simulink model "s_b4a4x4kf"  (R2018a)
settings: Solver=VariableStepDiscrete  StartTime=0.0  StopTime=1  RelTol=1e-3
undefined symbols (not defined in the file): fft_stages, n_bits_ants, n_bits_xengs
libraries: xbsIndex_r4 x22457, casper_library_misc x31, xbsReplacements_r4 x30, casper_library_scopes x17, xps_library x4
(part 141 of 232)

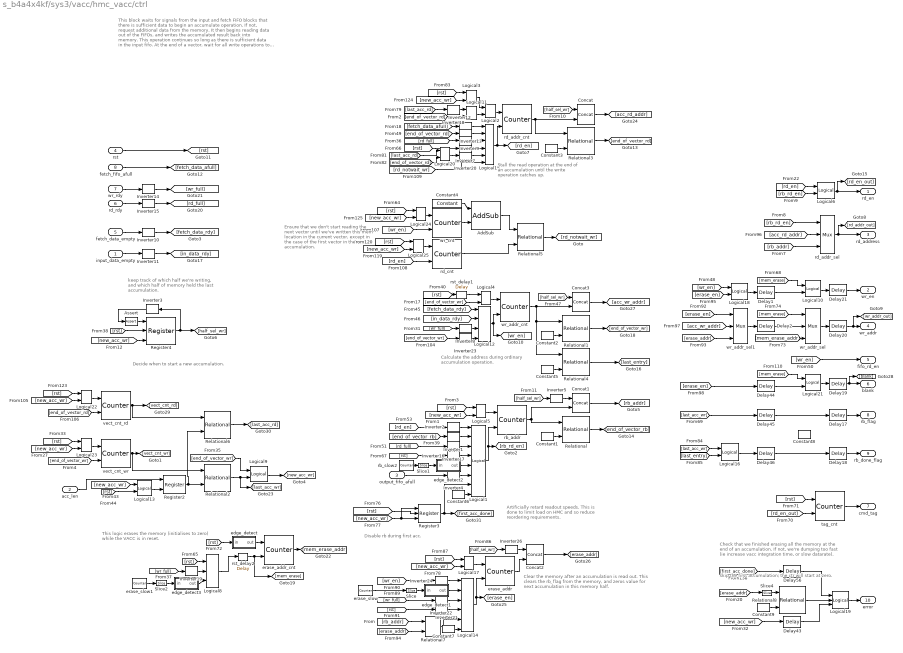
== system s_b4a4x4kf/sys3/vacc/hmc_vacc/ctrl ==
  note: Clear the memory after an accumulation is read out.
      | This clears the rb_flag from the memory, and
      | zeros value for next accumulation in this memory half.
  note: Stall the read operation
      | at the end of an accumulation
      | until the write operation catches up.
  note: Ensure that we don't start reading
      | the next vector until we've written
      | this mem location in the current vector,
      | except in the case of the first vector in
      | the accumulation.
  note: Disable rb during first acc.
  note: Artificially retard readout speeds.
      | This is done to limit load on HMC and
      | so reduce reordering requirements.
  note: This logic erases the memory (initialises to zero)
      | while the VACC is in reset.
  note: Decide when to start a new accumulation.
  note: Calculate the address during ordinary
      | accumulation operation.
  note: keep track of which half we're writing,
      | and which half of memory
      | held the last accumulation.
  note: This block waits for signals from the
      | input and fetch FIFO blocks that there is sufficient data
      | to begin an accumulate operation.
      |
      | If not, request additional data from the memory.
      |
      | It then begins reading data out of the FIFOs, and writes the
      | accumulated result back into memory.
      |
      | This operation continues so long as there is
      | sufficient data in the input fifo.
      |
      | At the end of a vector, wait for all write operations
      | to finish before starting the next vector.
      |
      | Simultaneously, read back the previous integration during
      | unused rd/write operations. After reading a previous accumulated
      | value, try to clear that memory location.
  note: Check that we finished erasing all the memory
      | at the end of an accumulation.
      | If not, we're dumping too fast
      | (ie increase vacc integration time, or slow datarate).
  note: skip the first accumulation; the ctr will start at zero.
  input_data_empty : Inport
  acc_len : Inport  Port=2
  output_fifo_afull : Inport  Port=3
  rst : Inport  Port=4
  fetch_data_empty : Inport  Port=5
  rd_rdy : Inport  Port=6
  wr_rdy : Inport  Port=7
  fetch_fifo_afull : Inport  Port=8
  AddSub : xbsIndex_r4/AddSub  mode=Addition  use_carryin=off  use_carryout=off  en=off  latency=1  precision=Full  arith_type=Unsigned  n_bits=16  bin_pt=14  quantization=Truncate  overflow=Wrap  use_behavioral_HDL=off  hw_selection=Fabric  pipelined=off  dbl_ovrd=off  block_type=addsub
  Assert : xbsIndex_r4/Assert  assert_type=on  type_source=Explicitly  gui_display_data_type=Fixed-point  arith_type=Unsigned  n_bits=1  bin_pt=0  preci_type=Single  exp_width=8  frac_width=24  assert_rate=on  rate_source=Explicitly  period=1  output_port=on  block_type=assert
      settings: infoedit=Asserts a user-defined sample rate and/or type on a signal.<P><P>Hardware notes: In hardware this block costs nothing.  block_version=10.1.3
  Concat{,1..3} (4 alike) : xbsIndex_r4/Concat  num_inputs=2  dbl_ovrd=off  block_type=concat
      settings: block_version=10.1.3
  Constant{1..3,9} (4 alike) : xbsIndex_r4/Constant  const=vector_len  gui_display_data_type=Fixed-point  arith_type=Unsigned  n_bits=vector_bits  bin_pt=0  preci_type=Single  exp_width=8  frac_width=24  explicit_period=on  period=1  equ=P=C  opselect=C  inp2=PCIN>>17  opr=+  inp1=P  carry=CIN  dbl_ovrd=off  block_type=constant
  Constant4 : xbsIndex_r4/Constant  const=vector_len-4  gui_display_data_type=Fixed-point  arith_type=Unsigned  n_bits=vector_bits  bin_pt=0  preci_type=Single  exp_width=8  frac_width=24  explicit_period=on  period=1  equ=P=C  opselect=C  inp2=PCIN>>17  opr=+  inp1=P  carry=CIN  dbl_ovrd=off  block_type=constant
  Constant5 : xbsIndex_r4/Constant  const=vector_len-1  gui_display_data_type=Fixed-point  arith_type=Unsigned  n_bits=vector_bits  bin_pt=0  preci_type=Single  exp_width=8  frac_width=24  explicit_period=on  period=1  equ=P=C  opselect=C  inp2=PCIN>>17  opr=+  inp1=P  carry=CIN  dbl_ovrd=off  block_type=constant
  Constant6 : xbsIndex_r4/Constant  const=1  gui_display_data_type=Boolean  arith_type=Boolean  n_bits=1  bin_pt=0  preci_type=Single  exp_width=8  frac_width=24  explicit_period=on  period=1  equ=P=C  opselect=C  inp2=PCIN>>17  opr=+  inp1=P  carry=CIN  dbl_ovrd=off  block_type=constant
  Constant7 : xbsIndex_r4/Constant  const=1  gui_display_data_type=Boolean  arith_type=Boolean  n_bits=1  bin_pt=0  preci_type=Single  exp_width=8  frac_width=24  explicit_period=on  period=1  equ=P=C  opselect=C  inp2=PCIN>>17  opr=+  inp1=P  carry=CIN  dbl_ovrd=off  block_type=constant
  Constant8 : xbsIndex_r4/Constant  const=0  gui_display_data_type=Boolean  arith_type=Boolean  n_bits=1  bin_pt=0  preci_type=Single  exp_width=8  frac_width=24  explicit_period=on  period=1  equ=P=C  opselect=C  inp2=PCIN>>17  opr=+  inp1=P  carry=CIN  dbl_ovrd=off  block_type=constant
  Delay{1..2,44..46} (5 alike) : xbsIndex_r4/Delay  rst=off  infoeditControl=Selection of Reset will increase slice count due to use of real FFs and instead of SRLs  en=off  latency=delay_fifo  reg_retiming=on  dbl_ovrd=off  block_type=delay
      settings: infoedit=Hardware notes: A delay line is a chain, each link of which is an SRL16 or SRL32 followed by a flip-flop.
  Delay{17..21} (5 alike) : xbsIndex_r4/Delay  rst=off  infoeditControl=Selection of Reset will increase slice count due to use of real FFs and instead of SRLs  en=off  latency=delay_adder  reg_retiming=on  dbl_ovrd=off  block_type=delay
      settings: infoedit=Hardware notes: A delay line is a chain, each link of which is an SRL16 or SRL32 followed by a flip-flop.
  Delay43 : xbsIndex_r4/Delay  rst=off  infoeditControl=Selection of Reset will increase slice count due to use of real FFs and instead of SRLs  en=off  latency=1  reg_retiming=on  dbl_ovrd=off  block_type=delay
      settings: infoedit=Hardware notes: A delay line is a chain, each link of which is an SRL16 or SRL32 followed by a flip-flop.
  Delay56 : xbsIndex_r4/Delay  rst=off  infoeditControl=Selection of Reset will increase slice count due to use of real FFs and instead of SRLs  en=off  latency=1  reg_retiming=on  dbl_ovrd=off  block_type=delay
      settings: infoedit=Hardware notes: A delay line is a chain, each link of which is an SRL16 or SRL32 followed by a flip-flop.
  Inverter{1..5,7..24,26} (24 alike) : xbsIndex_r4/Inverter  en=off  latency=0  dbl_ovrd=off  block_type=inv
  Logical1 : xbsIndex_r4/Logical  logical_function=AND  inputs=8  en=off  latency=0  precision=Full  arith_type=Unsigned  n_bits=16  bin_pt=0  align_bp=on  dbl_ovrd=off  block_type=logical
  Logical{2..6,10,13,17..18,21..25} (14 alike) : xbsIndex_r4/Logical  logical_function=OR  inputs=2  en=off  latency=0  precision=Full  arith_type=Unsigned  n_bits=16  bin_pt=0  align_bp=on  dbl_ovrd=off  block_type=logical
  Logical{9,11,16,20} (4 alike) : xbsIndex_r4/Logical  logical_function=AND  inputs=2  en=off  latency=0  precision=Full  arith_type=Unsigned  n_bits=16  bin_pt=0  align_bp=on  dbl_ovrd=off  block_type=logical
  Logical12 : xbsIndex_r4/Logical  logical_function=AND  inputs=4  en=off  latency=0  precision=Full  arith_type=Unsigned  n_bits=16  bin_pt=0  align_bp=on  dbl_ovrd=off  block_type=logical
  Logical14 : xbsIndex_r4/Logical  logical_function=AND  inputs=6  en=off  latency=0  precision=Full  arith_type=Unsigned  n_bits=16  bin_pt=0  align_bp=on  dbl_ovrd=off  block_type=logical
  Logical15 : xbsIndex_r4/Logical  logical_function=AND  inputs=6  en=off  latency=0  precision=Full  arith_type=Unsigned  n_bits=16  bin_pt=0  align_bp=on  dbl_ovrd=off  block_type=logical
  Logical19 : xbsIndex_r4/Logical  logical_function=AND  inputs=3  en=off  latency=0  precision=Full  arith_type=Unsigned  n_bits=16  bin_pt=0  align_bp=on  dbl_ovrd=off  block_type=logical
  Logical8 : xbsIndex_r4/Logical  logical_function=AND  inputs=3  en=off  latency=0  precision=Full  arith_type=Unsigned  n_bits=16  bin_pt=0  align_bp=on  dbl_ovrd=off  block_type=logical
  Register2 : xbsIndex_r4/Register  init=0  rst=off  en=on  dbl_ovrd=off  block_type=register
  Register3 : xbsIndex_r4/Register  init=0  rst=on  en=on  dbl_ovrd=off  block_type=register
  Register4 : xbsIndex_r4/Register  init=0  rst=on  en=on  dbl_ovrd=off  block_type=register
  Relational{,1..4,6} (6 alike) : xbsIndex_r4/Relational  mode=a>=b  op_type=Bool  en=off  latency=0  dbl_ovrd=off  block_type=relational
      settings: block_version=10.1.3
  Relational5 : xbsIndex_r4/Relational  mode=a>b  op_type=Bool  en=off  latency=1  dbl_ovrd=off  block_type=relational
      settings: block_version=10.1.3
  Relational7 : xbsIndex_r4/Relational  mode=a>b  op_type=Bool  en=off  latency=0  dbl_ovrd=off  block_type=relational
      settings: block_version=10.1.3
  Relational8 : xbsIndex_r4/Relational  mode=a!=b  op_type=Bool  en=off  latency=1  dbl_ovrd=off  block_type=relational
      settings: block_version=10.1.3
  Slice : xbsIndex_r4/Slice  nbits=1  boolean_output=on  mode=Upper Bit Location + Width  bit1=0  base1=MSB of Input  bit0=0  base0=LSB of Input  dbl_ovrd=off  block_type=slice
  Slice1 : xbsIndex_r4/Slice  nbits=1  boolean_output=on  mode=Upper Bit Location + Width  bit1=0  base1=MSB of Input  bit0=0  base0=LSB of Input  dbl_ovrd=off  block_type=slice
  Slice2 : xbsIndex_r4/Slice  nbits=1  boolean_output=on  mode=Upper Bit Location + Width  bit1=0  base1=MSB of Input  bit0=0  base0=LSB of Input  dbl_ovrd=off  block_type=slice
  Slice4 : xbsIndex_r4/Slice  nbits=1  boolean_output=off  mode=Two Bit Locations  bit1=-1  base1=MSB of Input  bit0=0  base0=LSB of Input  dbl_ovrd=off  block_type=slice
  edge_detect : Subsystem  mask(edge_detect){edge=Rising, polarity=Active High, x_in=[0 0.08 0.08 0.16 0.16 0.24 0.24 0.32 0.32 0.4], y_in=[-1 -1  1  1  1  1  1  1  1  1], x_out=[0.6 0.68 0.68 0.76 0.76 0.84 0.84 0.92 0.92 1], y_out=[-1 -1  1  1 -1 -1 -1 -1 -1 -1]}
      mask prompts: edge "Edge Type"; polarity "Output Polarity"; x_in "Input X Positions"; y_in "Input Y Positions"; x_out "Output X Positions"; y_out "Output Y Positions"
      mask help: Output is active for one-cycle after each edge of the specified type (i.e. rising, falling or both).
      mask init: same as s_b4a4x4kf/edge_detect
      settings: AttributesFormatString=|
      | rising edges
      | active high
      mask Help: Output is active for one-cycle after each edge of the specified type (i.e. rising, falling, or both).  Latency is zero.
      mask TypeOptions edge: Rising | Falling | Both
      mask TypeOptions polarity: Active High | Active Low
      mask Display:
      | plot(x_in_num,0.5+y_in_num*0.2);
      | plot(x_out_num,0.5+y_out_num*0.2);
  edge_detect1 : Subsystem  mask(edge_detect){edge=Rising, polarity=Active High, x_in=[0 0.08 0.08 0.16 0.16 0.24 0.24 0.32 0.32 0.4], y_in=[-1 -1  1  1  1  1  1  1  1  1], x_out=[0.6 0.68 0.68 0.76 0.76 0.84 0.84 0.92 0.92 1], y_out=[-1 -1  1  1 -1 -1 -1 -1 -1 -1]}
      mask prompts: edge "Edge Type"; polarity "Output Polarity"; x_in "Input X Positions"; y_in "Input Y Positions"; x_out "Output X Positions"; y_out "Output Y Positions"
      mask help: Output is active for one-cycle after each edge of the specified type (i.e. rising, falling or both).
      mask init: same as s_b4a4x4kf/edge_detect
      settings: AttributesFormatString=|
      | rising edges
      | active high
      mask Help: Output is active for one-cycle after each edge of the specified type (i.e. rising, falling, or both).  Latency is zero.
      mask TypeOptions edge: Rising | Falling | Both
      mask TypeOptions polarity: Active High | Active Low
      mask Display:
      | plot(x_in_num,0.5+y_in_num*0.2);
      | plot(x_out_num,0.5+y_out_num*0.2);
  edge_detect2 : Subsystem  mask(edge_detect){edge=Rising, polarity=Active High, x_in=[0 0.08 0.08 0.16 0.16 0.24 0.24 0.32 0.32 0.4], y_in=[-1 -1  1  1  1  1  1  1  1  1], x_out=[0.6 0.68 0.68 0.76 0.76 0.84 0.84 0.92 0.92 1], y_out=[-1 -1  1  1 -1 -1 -1 -1 -1 -1]}
      mask prompts: edge "Edge Type"; polarity "Output Polarity"; x_in "Input X Positions"; y_in "Input Y Positions"; x_out "Output X Positions"; y_out "Output Y Positions"
      mask help: Output is active for one-cycle after each edge of the specified type (i.e. rising, falling or both).
      mask init: same as s_b4a4x4kf/edge_detect
      settings: AttributesFormatString=|
      | rising edges
      | active high
      mask Help: Output is active for one-cycle after each edge of the specified type (i.e. rising, falling, or both).  Latency is zero.
      mask TypeOptions edge: Rising | Falling | Both
      mask TypeOptions polarity: Active High | Active Low
      mask Display:
      | plot(x_in_num,0.5+y_in_num*0.2);
      | plot(x_out_num,0.5+y_out_num*0.2);
  edge_detect3 : Subsystem  mask(edge_detect){edge=Rising, polarity=Active High, x_in=[0 0.08 0.08 0.16 0.16 0.24 0.24 0.32 0.32 0.4], y_in=[-1 -1  1  1  1  1  1  1  1  1], x_out=[0.6 0.68 0.68 0.76 0.76 0.84 0.84 0.92 0.92 1], y_out=[-1 -1  1  1 -1 -1 -1 -1 -1 -1]}
      mask prompts: edge "Edge Type"; polarity "Output Polarity"; x_in "Input X Positions"; y_in "Input Y Positions"; x_out "Output X Positions"; y_out "Output Y Positions"
      mask help: Output is active for one-cycle after each edge of the specified type (i.e. rising, falling or both).
      mask init: same as s_b4a4x4kf/edge_detect
      settings: AttributesFormatString=|
      | rising edges
      | active high
      mask Help: Output is active for one-cycle after each edge of the specified type (i.e. rising, falling, or both).  Latency is zero.
      mask TypeOptions edge: Rising | Falling | Both
      mask TypeOptions polarity: Active High | Active Low
      mask Display:
      | plot(x_in_num,0.5+y_in_num*0.2);
      | plot(x_out_num,0.5+y_out_num*0.2);
  erase_addr : xbsIndex_r4/Counter  cnt_type=Free Running  cnt_to=Inf  operation=Up  start_count=0  cnt_by_val=1  arith_type=Unsigned  n_bits=vector_bits  bin_pt=0  load_pin=off  rst=on  en=on  explicit_period=on  period=1  use_behavioral_HDL=off  implementation=Fabric  use_rpm=off  dbl_ovrd=off  block_type=counter
  erase_addr_cnt : xbsIndex_r4/Counter  cnt_type=Free Running  cnt_to=vector_len-1  operation=Up  start_count=0  cnt_by_val=1  arith_type=Unsigned  n_bits=vector_bits+1  bin_pt=0  load_pin=off  rst=on  en=on  explicit_period=on  period=1  use_behavioral_HDL=off  implementation=Fabric  use_rpm=off  dbl_ovrd=off  block_type=counter
  erase_slow : xbsIndex_r4/Counter  cnt_type=Free Running  cnt_to=Inf  operation=Up  start_count=0  cnt_by_val=1  arith_type=Unsigned  n_bits=4  bin_pt=0  load_pin=off  rst=off  en=off  explicit_period=on  period=1  use_behavioral_HDL=on  implementation=Fabric  use_rpm=off  dbl_ovrd=off  block_type=counter
  erase_slow1 : xbsIndex_r4/Counter  cnt_type=Free Running  cnt_to=Inf  operation=Up  start_count=0  cnt_by_val=1  arith_type=Unsigned  n_bits=2  bin_pt=0  load_pin=off  rst=off  en=off  explicit_period=on  period=1  use_behavioral_HDL=on  implementation=Fabric  use_rpm=off  dbl_ovrd=off  block_type=counter
  rb_addr : xbsIndex_r4/Counter  cnt_type=Free Running  cnt_to=Inf  operation=Up  start_count=0  cnt_by_val=1  arith_type=Unsigned  n_bits=vector_bits  bin_pt=0  load_pin=off  rst=on  en=on  explicit_period=on  period=1  use_behavioral_HDL=off  implementation=Fabric  use_rpm=off  dbl_ovrd=off  block_type=counter
  rb_slow2 : xbsIndex_r4/Counter  cnt_type=Free Running  cnt_to=Inf  operation=Up  start_count=0  cnt_by_val=1  arith_type=Unsigned  n_bits=4  bin_pt=0  load_pin=off  rst=off  en=off  explicit_period=on  period=1  use_behavioral_HDL=on  implementation=Fabric  use_rpm=off  dbl_ovrd=off  block_type=counter
  rd_addr_cnt : xbsIndex_r4/Counter  cnt_type=Free Running  cnt_to=vector_len-1  operation=Up  start_count=0  cnt_by_val=1  arith_type=Unsigned  n_bits=vector_bits  bin_pt=0  load_pin=off  rst=on  en=on  explicit_period=on  period=1  use_behavioral_HDL=off  implementation=Fabric  use_rpm=off  dbl_ovrd=off  block_type=counter
  rd_addr_sel : xbsIndex_r4/Mux  inputs=2  en=off  latency=0  precision=Full  arith_type=Unsigned  n_bits=16  bin_pt=14  quantization=Truncate  overflow=Wrap  dbl_ovrd=off  block_type=mux
  rd_cnt : xbsIndex_r4/Counter  cnt_type=Free Running  cnt_to=vector_len-1  operation=Up  start_count=0  cnt_by_val=1  arith_type=Unsigned  n_bits=vector_bits+22  bin_pt=0  load_pin=off  rst=on  en=on  explicit_period=on  period=1  use_behavioral_HDL=off  implementation=Fabric  use_rpm=off  dbl_ovrd=off  block_type=counter
  rst_delay1 : xbsIndex_r4/Delay  rst=off  infoeditControl=Selection of Reset will increase slice count due to use of real FFs and instead of SRLs  en=off  latency=2  reg_retiming=on  dbl_ovrd=off  block_type=delay
  rst_delay2 : xbsIndex_r4/Delay  rst=off  infoeditControl=Selection of Reset will increase slice count due to use of real FFs and instead of SRLs  en=off  latency=1  reg_retiming=on  dbl_ovrd=off  block_type=delay
      settings: infoedit=Hardware notes: A delay line is a chain, each link of which is an SRL16 or SRL32 followed by a flip-flop.
  tag_cnt : xbsIndex_r4/Counter  cnt_type=Free Running  cnt_to=Inf  operation=Up  start_count=0  cnt_by_val=1  arith_type=Unsigned  n_bits=9  bin_pt=0  load_pin=off  rst=on  en=on  explicit_period=on  period=1  use_behavioral_HDL=off  implementation=Fabric  use_rpm=off  dbl_ovrd=off  block_type=counter
  vect_cnt_rd : xbsIndex_r4/Counter  cnt_type=Free Running  cnt_to=Inf  operation=Up  start_count=1  cnt_by_val=1  arith_type=Unsigned  n_bits=32  bin_pt=0  load_pin=off  rst=on  en=on  explicit_period=on  period=1  use_behavioral_HDL=off  implementation=Fabric  use_rpm=off  dbl_ovrd=off  block_type=counter
  vect_cnt_wr : xbsIndex_r4/Counter  cnt_type=Free Running  cnt_to=Inf  operation=Up  start_count=1  cnt_by_val=1  arith_type=Unsigned  n_bits=32  bin_pt=0  load_pin=off  rst=on  en=on  explicit_period=on  period=1  use_behavioral_HDL=off  implementation=Fabric  use_rpm=off  dbl_ovrd=off  block_type=counter
  wr_addr_cnt : xbsIndex_r4/Counter  cnt_type=Free Running  cnt_to=vector_len-1  operation=Up  start_count=0  cnt_by_val=1  arith_type=Unsigned  n_bits=vector_bits  bin_pt=0  load_pin=off  rst=on  en=on  explicit_period=on  period=1  use_behavioral_HDL=off  implementation=Fabric  use_rpm=off  dbl_ovrd=off  block_type=counter
  wr_addr_sel : xbsIndex_r4/Mux  inputs=2  en=off  latency=0  precision=Full  arith_type=Unsigned  n_bits=16  bin_pt=14  quantization=Truncate  overflow=Wrap  dbl_ovrd=off  block_type=mux
  wr_addr_sel1 : xbsIndex_r4/Mux  inputs=2  en=off  latency=0  precision=Full  arith_type=Unsigned  n_bits=16  bin_pt=14  quantization=Truncate  overflow=Wrap  dbl_ovrd=off  block_type=mux
  wr_cnt : xbsIndex_r4/Counter  cnt_type=Free Running  cnt_to=vector_len-1  operation=Up  start_count=0  cnt_by_val=1  arith_type=Unsigned  n_bits=vector_bits+22  bin_pt=0  load_pin=off  rst=on  en=on  explicit_period=on  period=1  use_behavioral_HDL=off  implementation=Fabric  use_rpm=off  dbl_ovrd=off  block_type=counter
  rd_en : Outport
  wr_en : Outport  Port=2
  rd_address : Outport  Port=3
  wr_addr : Outport  Port=4
  fifo_rd_en : Outport  Port=5
  blank : Outport  Port=6
  cmd_tag : Outport  Port=7
  rb_flag : Outport  Port=8
  rb_done_flag : Outport  Port=9
  error : Outport  Port=10
  wires:
  Concat1/1 -> [rb_addr]
  rb_addr/1 -> Concat1/2, Relational/1
  [rb_addr] -> rd_addr_sel/3
  Inverter5/1 -> Concat1/1
  [half_sel_wr] -> Inverter5/1
  [half_sel_wr] -> Concat/1
  Register2/1 -> Relational6/2, Relational2/2
  Logical9/1 -> [new_acc_wr]
  rst/1 -> [rst]
  Constant3/1 -> Relational3/2
  Assert/1 -> Register4/1
  Inverter3/1 -> Assert/1
  Register4/1 -> [half_sel_wr], Inverter3/1
  rd_addr_sel/1 -> rd_address/1, [rd_addr_out]
  [rb_rd_en] -> Logical6/2
  Concat/1 -> [acc_rd_addr]
  [rb_rd_en] -> rd_addr_sel/1
  Logical6/1 -> rd_en/1, [rd_en_out]
  Relational/1 -> [end_of_vector_rb]
  rd_addr_cnt/1 -> Relational3/1, Concat/2
  Logical15/1 -> rd_addr_cnt/2, [rd_en]
  [end_of_vector_wr] -> vect_cnt_wr/2
  Logical2/1 -> rd_addr_cnt/1
  Logical3/1 -> Logical2/1
  Relational2/1 -> [last_acc_wr], Logical9/2
  [end_of_vector_wr] -> Logical9/1
  Logical1/1 -> rb_addr/2, [rb_rd_en]
  [rst] -> Register4/2
  [rd_en] -> Inverter2/1
  [new_acc_wr] -> Logical13/1
  [rst] -> Logical13/2
  acc_len/1 -> Register2/1
  Logical13/1 -> Register2/2
  Logical4/1 -> wr_addr_cnt/1
  fetch_data_empty/1 -> Inverter10/1
  input_data_empty/1 -> Inverter11/1
  Inverter10/1 -> [fetch_data_rdy]
  Inverter11/1 -> [in_data_rdy]
  [fetch_data_afull] -> Inverter12/1
  [end_of_vector_rd] -> Inverter13/1
  Inverter12/1 -> Logical15/1
  Inverter13/1 -> Logical15/2
  Relational1/1 -> [end_of_vector_wr]
  Constant2/1 -> Relational1/2
  [end_of_vector_wr] -> Logical4/2
  [rst] -> rst_delay1/1
  [fetch_data_rdy] -> Logical12/1
  [in_data_rdy] -> Logical12/2
  Logical12/1 -> wr_addr_cnt/2, [wr_en]
  [half_sel_wr] -> Concat3/1
  wr_addr_cnt/1 -> Concat3/2, Relational1/1, Relational4/1
  [rd_en] -> Logical6/1
  [wr_en] -> fifo_rd_en/1
  Constant1/1 -> Relational/2
  [end_of_vector_rb] -> Inverter1/1
  rd_rdy/1 -> Inverter15/1
  wr_rdy/1 -> Inverter14/1
  [wr_full] -> Inverter8/1
  Inverter8/1 -> Logical12/3
  [rd_full] -> Inverter9/1
  Inverter14/1 -> [wr_full]
  Inverter15/1 -> [rd_full]
  Delay2/1 -> wr_addr_sel/2
  [rd_full] -> Inverter17/1
  output_fifo_afull/1 -> Inverter4/1
  fetch_fifo_afull/1 -> [fetch_data_afull]
  Inverter17/1 -> Logical1/3
  Inverter2/1 -> Logical1/1
  Inverter1/1 -> Logical1/2
  Inverter9/1 -> Logical15/3
  Constant5/1 -> Relational4/2
  Relational4/1 -> [last_entry]
  [new_acc_wr] -> Logical5/2
  [rst] -> Logical5/1
  Logical5/1 -> rb_addr/1
  [rst] -> Inverter7/1
  Inverter7/1 -> Logical15/4
  [rst] -> Inverter16/1
  edge_detect2/1(out) -> Logical1/5
  Inverter16/1 -> Logical1/4
  [rd_en_out] -> tag_cnt/2
  tag_cnt/1 -> cmd_tag/1
  rst_delay1/1 -> Logical4/1
  [rst] -> Logical8/1
  [wr_full] -> Inverter19/1
  Inverter19/1 -> Logical8/2
  Logical8/1 -> rst_delay2/1
  rst_delay2/1 -> erase_addr_cnt/2, [mem_erase]
  [rst] -> edge_detect/1(in)
  edge_detect/1(out) -> erase_addr_cnt/1
  wr_addr_sel/1 -> Delay20/1
  erase_addr_cnt/1 -> [mem_erase_addr]
  [mem_erase_addr] -> wr_addr_sel/3
  [mem_erase] -> wr_addr_sel/1
  Logical10/1 -> Delay21/1
  Delay1/1 -> Logical10/2
  [mem_erase] -> Logical10/1
  Inverter4/1 -> Logical1/6
  [rst] -> Register3/2
  [new_acc_wr] -> Register3/3, Register3/1
  vect_cnt_wr/1 -> Relational2/1, [vect_cnt_wr]
  [last_acc_wr] -> Logical16/1
  [last_entry] -> Logical16/2
  Delay17/1 -> rb_flag/1
  Delay18/1 -> rb_done_flag/1
  Concat2/1 -> [erase_addr]
  erase_addr/1 -> Concat2/2
  Inverter26/1 -> Concat2/1
  [half_sel_wr] -> Inverter26/1
  Logical14/1 -> [erase_en], erase_addr/2
  [wr_en] -> Inverter24/1
  [wr_full] -> Inverter22/1
  Inverter22/1 -> Logical14/3
  Inverter24/1 -> Logical14/1
  [new_acc_wr] -> Logical17/2
  [rst] -> Logical17/1
  Logical17/1 -> erase_addr/1
  [rst] -> Inverter21/1
  Relational7/1 -> Logical14/5
  Inverter21/1 -> Logical14/4
  Slice/1 -> edge_detect1/1(in)
  [rb_addr] -> Relational7/1
  [erase_addr] -> Relational7/2
  wr_addr_sel1/1 -> Delay2/1
  [erase_en] -> wr_addr_sel1/1
  [erase_addr] -> wr_addr_sel1/3
  edge_detect1/1(out) -> Logical14/2
  [wr_en] -> Logical18/1
  [erase_en] -> Logical18/2
  Logical18/1 -> Delay1/1
  [acc_rd_addr] -> rd_addr_sel/2
  Concat3/1 -> [acc_wr_addr]
  [acc_wr_addr] -> wr_addr_sel1/2
  [erase_en] -> Delay44/1
  Register3/1 -> [first_acc_done], Logical1/7
  Delay20/1 -> wr_addr/1, [wr_addr_out]
  Delay21/1 -> wr_en/1
  rb_slow2/1 -> Slice1/1
  Slice1/1 -> edge_detect2/1(in)
  [last_acc_rd] -> Inverter18/1
  Inverter18/1 -> Logical11/1
  [end_of_vector_rd] -> Logical11/2
  Logical11/1 -> Logical2/2
  [end_of_vector_rd] -> Logical20/2
  [last_acc_rd] -> Logical20/1
  Logical20/1 -> Inverter20/1
  Inverter20/1 -> Logical15/5
  [end_of_vector_wr] -> Inverter23/1
  Inverter23/1 -> Logical12/4
  erase_slow/1 -> Slice/1
  Slice2/1 -> edge_detect3/1(in)
  erase_slow1/1 -> Slice2/1
  edge_detect3/1(out) -> Logical8/3
  Relational3/1 -> [end_of_vector_rd]
  [rd_notwait_wr] -> Logical15/6
  rd_cnt/1 -> Relational5/2
  Relational5/1 -> [rd_notwait_wr]
  Logical25/1 -> rd_cnt/1
  Logical24/1 -> wr_cnt/1
  [wr_en] -> wr_cnt/2
  [rd_en] -> rd_cnt/2
  wr_cnt/1 -> AddSub/2
  Constant4/1 -> AddSub/1
  AddSub/1 -> Relational5/1
  Logical22/1 -> vect_cnt_rd/1
  vect_cnt_rd/1 -> Relational6/1, [vect_cnt_rd]
  [end_of_vector_rd] -> vect_cnt_rd/2
  Relational6/1 -> [last_acc_rd]
  [new_acc_wr] -> Logical22/2
  [rst] -> Logical22/1
  [new_acc_wr] -> Logical3/2
  [rst] -> Logical3/1
  Constant6/1 -> Logical1/8
  Constant7/1 -> Logical14/6
  [rst] -> tag_cnt/1
  [new_acc_wr] -> Logical23/2
  [rst] -> Logical23/1
  Logical23/1 -> vect_cnt_wr/1
  Logical16/1 -> Delay46/1
  [new_acc_wr] -> Logical24/2
  [rst] -> Logical24/1
  [new_acc_wr] -> Logical25/2
  [rst] -> Logical25/1
  [new_acc_wr] -> Register4/3
  Delay19/1 -> blank/1, [blank]
  [last_acc_wr] -> Delay45/1
  Delay45/1 -> Delay17/1
  Delay46/1 -> Delay18/1
  [mem_erase] -> Logical21/1
  Logical21/1 -> Delay19/1
  Delay44/1 -> Logical21/2
  [new_acc_wr] -> Delay43/1
  [erase_addr] -> Slice4/1
  Relational8/1 -> Logical19/2
  Constant9/1 -> Relational8/2
  Delay43/1 -> Logical19/3
  [first_acc_done] -> Delay56/1
  Slice4/1 -> Relational8/1
  Delay56/1 -> Logical19/1
  Logical19/1 -> error/1

== system s_b4a4x4kf/sys3/vacc/hmc_vacc/fifo_out_cnt ==
  out_reg : Inport
  assert_reg : xbsIndex_r4/Assert  assert_type=on  type_source=Explicitly  gui_display_data_type=Fixed-point  arith_type=Unsigned  n_bits=32  bin_pt=0  preci_type=Single  exp_width=8  frac_width=24  assert_rate=off  rate_source=Explicitly  period=1  output_port=on  block_type=assert
  cast_gw : xbsIndex_r4/Convert  gui_display_data_type=Fixed-point  arith_type=Unsigned  n_bits=32  bin_pt=0  float_type=Single  exp_bits=8  fraction_bits=24  quantization=Truncate  overflow=Wrap  en=off  latency=1  pipeline=off  dbl_ovrd=off  block_type=convert
  io_delay : xbsIndex_r4/Delay  rst=off  infoeditControl=Selection of Reset will increase slice count due to use of real FFs and instead of SRLs  en=off  latency=0  reg_retiming=on  dbl_ovrd=off  block_type=delay
  reint1 : xbsIndex_r4/Reinterpret  force_arith_type=on  arith_type=Unsigned  force_bin_pt=on  bin_pt=0  block_type=reinterpret
  s_b4a4x4kf_sys3_vacc_hmc_vacc_fifo_out_cnt_user_data_in : xbsIndex_r4/Gateway Out  inherit_from_input=off  hdl_port=on  rows=1  columns=1  UseAsDAC=off  DACChannel='1'  interface=None  automatic_assignment=on  address_offset=hex2dec('00')  intf_name=''  intf_description=''  timing_constraint=None  locs_specified=off  LOCs={}  io_standard={}  block_type=gatewayout
  sim_out : Terminator
  wires:
  io_delay/1 -> cast_gw/1
  cast_gw/1 -> s_b4a4x4kf_sys3_vacc_hmc_vacc_fifo_out_cnt_user_data_in/1
  s_b4a4x4kf_sys3_vacc_hmc_vacc_fifo_out_cnt_user_data_in/1 -> sim_out/1
  out_reg/1 -> assert_reg/1
  assert_reg/1 -> reint1/1
  reint1/1 -> io_delay/1

== system s_b4a4x4kf/sys3/vacc/hmc_vacc/fifo_rd_cnt ==
  out_reg : Inport
  assert_reg : xbsIndex_r4/Assert  assert_type=on  type_source=Explicitly  gui_display_data_type=Fixed-point  arith_type=Unsigned  n_bits=32  bin_pt=0  preci_type=Single  exp_width=8  frac_width=24  assert_rate=off  rate_source=Explicitly  period=1  output_port=on  block_type=assert
  cast_gw : xbsIndex_r4/Convert  gui_display_data_type=Fixed-point  arith_type=Unsigned  n_bits=32  bin_pt=0  float_type=Single  exp_bits=8  fraction_bits=24  quantization=Truncate  overflow=Wrap  en=off  latency=1  pipeline=off  dbl_ovrd=off  block_type=convert
  io_delay : xbsIndex_r4/Delay  rst=off  infoeditControl=Selection of Reset will increase slice count due to use of real FFs and instead of SRLs  en=off  latency=0  reg_retiming=on  dbl_ovrd=off  block_type=delay
  reint1 : xbsIndex_r4/Reinterpret  force_arith_type=on  arith_type=Unsigned  force_bin_pt=on  bin_pt=0  block_type=reinterpret
  s_b4a4x4kf_sys3_vacc_hmc_vacc_fifo_rd_cnt_user_data_in : xbsIndex_r4/Gateway Out  inherit_from_input=off  hdl_port=on  rows=1  columns=1  UseAsDAC=off  DACChannel='1'  interface=None  automatic_assignment=on  address_offset=hex2dec('00')  intf_name=''  intf_description=''  timing_constraint=None  locs_specified=off  LOCs={}  io_standard={}  block_type=gatewayout
  sim_out : Terminator
  wires:
  io_delay/1 -> cast_gw/1
  cast_gw/1 -> s_b4a4x4kf_sys3_vacc_hmc_vacc_fifo_rd_cnt_user_data_in/1
  s_b4a4x4kf_sys3_vacc_hmc_vacc_fifo_rd_cnt_user_data_in/1 -> sim_out/1
  out_reg/1 -> assert_reg/1
  assert_reg/1 -> reint1/1
  reint1/1 -> io_delay/1

== system s_b4a4x4kf/sys3/vacc/hmc_vacc/fifo_status ==
  out_fetch_valid : Inport
  out_fetch_empty : Inport  Port=2
  out_fetch_full : Inport  Port=3
  out_fetch_afull : Inport  Port=4
  out_rst : Inport  Port=5
  out_fifo_rd_en : Inport  Port=6
  out_rb_en : Inport  Port=7
  out_out_ack : Inport  Port=8
  out_output_full : Inport  Port=9
  out_output_over : Inport  Port=10
  out_input_empty : Inport  Port=11
  out_input_over : Inport  Port=12
  out_output_empty : Inport  Port=13
  assert_fetch_afull : xbsIndex_r4/Assert  assert_type=on  type_source=Explicitly  gui_display_data_type=Boolean  arith_type=Boolean  n_bits=1  bin_pt=0  preci_type=Single  exp_width=8  frac_width=24  assert_rate=off  rate_source=Explicitly  period=1  output_port=on  block_type=assert
  assert_fetch_empty : xbsIndex_r4/Assert  assert_type=on  type_source=Explicitly  gui_display_data_type=Boolean  arith_type=Boolean  n_bits=1  bin_pt=0  preci_type=Single  exp_width=8  frac_width=24  assert_rate=off  rate_source=Explicitly  period=1  output_port=on  block_type=assert
  assert_fetch_full : xbsIndex_r4/Assert  assert_type=on  type_source=Explicitly  gui_display_data_type=Boolean  arith_type=Boolean  n_bits=1  bin_pt=0  preci_type=Single  exp_width=8  frac_width=24  assert_rate=off  rate_source=Explicitly  period=1  output_port=on  block_type=assert
  assert_fetch_valid : xbsIndex_r4/Assert  assert_type=on  type_source=Explicitly  gui_display_data_type=Boolean  arith_type=Boolean  n_bits=1  bin_pt=0  preci_type=Single  exp_width=8  frac_width=24  assert_rate=off  rate_source=Explicitly  period=1  output_port=on  block_type=assert
  assert_fifo_rd_en : xbsIndex_r4/Assert  assert_type=on  type_source=Explicitly  gui_display_data_type=Boolean  arith_type=Boolean  n_bits=1  bin_pt=0  preci_type=Single  exp_width=8  frac_width=24  assert_rate=off  rate_source=Explicitly  period=1  output_port=on  block_type=assert
  assert_input_empty : xbsIndex_r4/Assert  assert_type=on  type_source=Explicitly  gui_display_data_type=Boolean  arith_type=Boolean  n_bits=1  bin_pt=0  preci_type=Single  exp_width=8  frac_width=24  assert_rate=off  rate_source=Explicitly  period=1  output_port=on  block_type=assert
  assert_input_over : xbsIndex_r4/Assert  assert_type=on  type_source=Explicitly  gui_display_data_type=Boolean  arith_type=Boolean  n_bits=1  bin_pt=0  preci_type=Single  exp_width=8  frac_width=24  assert_rate=off  rate_source=Explicitly  period=1  output_port=on  block_type=assert
  assert_out_ack : xbsIndex_r4/Assert  assert_type=on  type_source=Explicitly  gui_display_data_type=Boolean  arith_type=Boolean  n_bits=1  bin_pt=0  preci_type=Single  exp_width=8  frac_width=24  assert_rate=off  rate_source=Explicitly  period=1  output_port=on  block_type=assert
  assert_output_empty : xbsIndex_r4/Assert  assert_type=on  type_source=Explicitly  gui_display_data_type=Boolean  arith_type=Boolean  n_bits=1  bin_pt=0  preci_type=Single  exp_width=8  frac_width=24  assert_rate=off  rate_source=Explicitly  period=1  output_port=on  block_type=assert
  assert_output_full : xbsIndex_r4/Assert  assert_type=on  type_source=Explicitly  gui_display_data_type=Boolean  arith_type=Boolean  n_bits=1  bin_pt=0  preci_type=Single  exp_width=8  frac_width=24  assert_rate=off  rate_source=Explicitly  period=1  output_port=on  block_type=assert
  assert_output_over : xbsIndex_r4/Assert  assert_type=on  type_source=Explicitly  gui_display_data_type=Boolean  arith_type=Boolean  n_bits=1  bin_pt=0  preci_type=Single  exp_width=8  frac_width=24  assert_rate=off  rate_source=Explicitly  period=1  output_port=on  block_type=assert
  assert_rb_en : xbsIndex_r4/Assert  assert_type=on  type_source=Explicitly  gui_display_data_type=Boolean  arith_type=Boolean  n_bits=1  bin_pt=0  preci_type=Single  exp_width=8  frac_width=24  assert_rate=off  rate_source=Explicitly  period=1  output_port=on  block_type=assert
  assert_rst : xbsIndex_r4/Assert  assert_type=on  type_source=Explicitly  gui_display_data_type=Boolean  arith_type=Boolean  n_bits=1  bin_pt=0  preci_type=Single  exp_width=8  frac_width=24  assert_rate=off  rate_source=Explicitly  period=1  output_port=on  block_type=assert
  cast_gw : xbsIndex_r4/Convert  gui_display_data_type=Fixed-point  arith_type=Unsigned  n_bits=32  bin_pt=0  float_type=Single  exp_bits=8  fraction_bits=24  quantization=Truncate  overflow=Wrap  en=off  latency=1  pipeline=off  dbl_ovrd=off  block_type=convert
  concatenate : xbsIndex_r4/Concat  num_inputs=13  dbl_ovrd=off  block_type=concat
  io_delay : xbsIndex_r4/Delay  rst=off  infoeditControl=Selection of Reset will increase slice count due to use of real FFs and instead of SRLs  en=off  latency=0  reg_retiming=on  dbl_ovrd=off  block_type=delay
  reint{1..13} (13 alike) : xbsIndex_r4/Reinterpret  force_arith_type=on  arith_type=Unsigned  force_bin_pt=on  bin_pt=0  block_type=reinterpret
  s_b4a4x4kf_sys3_vacc_hmc_vacc_fifo_status_user_data_in : xbsIndex_r4/Gateway Out  inherit_from_input=off  hdl_port=on  rows=1  columns=1  UseAsDAC=off  DACChannel='1'  interface=None  automatic_assignment=on  address_offset=hex2dec('00')  intf_name=''  intf_description=''  timing_constraint=None  locs_specified=off  LOCs={}  io_standard={}  block_type=gatewayout
  sim_out : Terminator
  wires:
  concatenate/1 -> io_delay/1
  io_delay/1 -> cast_gw/1
  cast_gw/1 -> s_b4a4x4kf_sys3_vacc_hmc_vacc_fifo_status_user_data_in/1
  s_b4a4x4kf_sys3_vacc_hmc_vacc_fifo_status_user_data_in/1 -> sim_out/1
  out_fetch_valid/1 -> assert_fetch_valid/1
  assert_fetch_valid/1 -> reint1/1
  reint1/1 -> concatenate/1
  out_fetch_empty/1 -> assert_fetch_empty/1
  assert_fetch_empty/1 -> reint2/1
  reint2/1 -> concatenate/2
  out_fetch_full/1 -> assert_fetch_full/1
  assert_fetch_full/1 -> reint3/1
  reint3/1 -> concatenate/3
  out_fetch_afull/1 -> assert_fetch_afull/1
  assert_fetch_afull/1 -> reint4/1
  reint4/1 -> concatenate/4
  out_rst/1 -> assert_rst/1
  assert_rst/1 -> reint5/1
  reint5/1 -> concatenate/5
  out_fifo_rd_en/1 -> assert_fifo_rd_en/1
  assert_fifo_rd_en/1 -> reint6/1
  reint6/1 -> concatenate/6
  out_rb_en/1 -> assert_rb_en/1
  assert_rb_en/1 -> reint7/1
  reint7/1 -> concatenate/7
  out_out_ack/1 -> assert_out_ack/1
  assert_out_ack/1 -> reint8/1
  reint8/1 -> concatenate/8
  out_output_full/1 -> assert_output_full/1
  assert_output_full/1 -> reint9/1
  reint9/1 -> concatenate/9
  out_output_over/1 -> assert_output_over/1
  assert_output_over/1 -> reint10/1
  reint10/1 -> concatenate/10
  out_input_empty/1 -> assert_input_empty/1
  assert_input_empty/1 -> reint11/1
  reint11/1 -> concatenate/11
  out_input_over/1 -> assert_input_over/1
  assert_input_over/1 -> reint12/1
  reint12/1 -> concatenate/12
  out_output_empty/1 -> assert_output_empty/1
  assert_output_empty/1 -> reint13/1
  reint13/1 -> concatenate/13

== system s_b4a4x4kf/sys3/vacc/hmc_vacc/fifo_wr_cnt ==
  out_reg : Inport
  assert_reg : xbsIndex_r4/Assert  assert_type=on  type_source=Explicitly  gui_display_data_type=Fixed-point  arith_type=Unsigned  n_bits=32  bin_pt=0  preci_type=Single  exp_width=8  frac_width=24  assert_rate=off  rate_source=Explicitly  period=1  output_port=on  block_type=assert
  cast_gw : xbsIndex_r4/Convert  gui_display_data_type=Fixed-point  arith_type=Unsigned  n_bits=32  bin_pt=0  float_type=Single  exp_bits=8  fraction_bits=24  quantization=Truncate  overflow=Wrap  en=off  latency=1  pipeline=off  dbl_ovrd=off  block_type=convert
  io_delay : xbsIndex_r4/Delay  rst=off  infoeditControl=Selection of Reset will increase slice count due to use of real FFs and instead of SRLs  en=off  latency=0  reg_retiming=on  dbl_ovrd=off  block_type=delay
  reint1 : xbsIndex_r4/Reinterpret  force_arith_type=on  arith_type=Unsigned  force_bin_pt=on  bin_pt=0  block_type=reinterpret
  s_b4a4x4kf_sys3_vacc_hmc_vacc_fifo_wr_cnt_user_data_in : xbsIndex_r4/Gateway Out  inherit_from_input=off  hdl_port=on  rows=1  columns=1  UseAsDAC=off  DACChannel='1'  interface=None  automatic_assignment=on  address_offset=hex2dec('00')  intf_name=''  intf_description=''  timing_constraint=None  locs_specified=off  LOCs={}  io_standard={}  block_type=gatewayout
  sim_out : Terminator
  wires:
  io_delay/1 -> cast_gw/1
  cast_gw/1 -> s_b4a4x4kf_sys3_vacc_hmc_vacc_fifo_wr_cnt_user_data_in/1
  s_b4a4x4kf_sys3_vacc_hmc_vacc_fifo_wr_cnt_user_data_in/1 -> sim_out/1
  out_reg/1 -> assert_reg/1
  assert_reg/1 -> reint1/1
  reint1/1 -> io_delay/1

== system s_b4a4x4kf/sys3/vacc/hmc_vacc/hmc_out_cnt ==
  out_reg : Inport
  assert_reg : xbsIndex_r4/Assert  assert_type=on  type_source=Explicitly  gui_display_data_type=Fixed-point  arith_type=Unsigned  n_bits=32  bin_pt=0  preci_type=Single  exp_width=8  frac_width=24  assert_rate=off  rate_source=Explicitly  period=1  output_port=on  block_type=assert
  cast_gw : xbsIndex_r4/Convert  gui_display_data_type=Fixed-point  arith_type=Unsigned  n_bits=32  bin_pt=0  float_type=Single  exp_bits=8  fraction_bits=24  quantization=Truncate  overflow=Wrap  en=off  latency=1  pipeline=off  dbl_ovrd=off  block_type=convert
  io_delay : xbsIndex_r4/Delay  rst=off  infoeditControl=Selection of Reset will increase slice count due to use of real FFs and instead of SRLs  en=off  latency=0  reg_retiming=on  dbl_ovrd=off  block_type=delay
  reint1 : xbsIndex_r4/Reinterpret  force_arith_type=on  arith_type=Unsigned  force_bin_pt=on  bin_pt=0  block_type=reinterpret
  s_b4a4x4kf_sys3_vacc_hmc_vacc_hmc_out_cnt_user_data_in : xbsIndex_r4/Gateway Out  inherit_from_input=off  hdl_port=on  rows=1  columns=1  UseAsDAC=off  DACChannel='1'  interface=None  automatic_assignment=on  address_offset=hex2dec('00')  intf_name=''  intf_description=''  timing_constraint=None  locs_specified=off  LOCs={}  io_standard={}  block_type=gatewayout
  sim_out : Terminator
  wires:
  io_delay/1 -> cast_gw/1
  cast_gw/1 -> s_b4a4x4kf_sys3_vacc_hmc_vacc_hmc_out_cnt_user_data_in/1
  s_b4a4x4kf_sys3_vacc_hmc_vacc_hmc_out_cnt_user_data_in/1 -> sim_out/1
  out_reg/1 -> assert_reg/1
  assert_reg/1 -> reint1/1
  reint1/1 -> io_delay/1

== system s_b4a4x4kf/sys3/vacc/hmc_vacc/hmc_pt2 ==
  In1 : Inport
  In2 : Inport  Port=2
  In3 : Inport  Port=3
  In4 : Inport  Port=4
  In5 : Inport  Port=5
  In6 : Inport  Port=6
  Out1 : Outport
  Out2 : Outport  Port=2
  Out3 : Outport  Port=3
  Out4 : Outport  Port=4
  Out5 : Outport  Port=5
  hmc_ok : Outport  Port=6
  tag scope: hmc1_1_data_in=global, hmc1_1_rd_addr=global, hmc1_1_rd_en=global, hmc1_1_tag_in=global, hmc1_1_wr_addr=global, hmc1_1_wr_en=global
  wires:
  In1/1 -> [hmc1_1_wr_en]
  [hmc1_ok] -> hmc_ok/1
  [hmc1_1_tag_out] -> Out4/1
  [hmc1_1_rd_rdy] -> Out5/1
  In2/1 -> [hmc1_1_wr_addr]
  In4/1 -> [hmc1_1_rd_en]
  In5/1 -> [hmc1_1_rd_addr]
  In3/1 -> [hmc1_1_data_in]
  In6/1 -> [hmc1_1_tag_in]
  [hmc1_1_wr_rdy] -> Out3/1
  [hmc1_1_data_out] -> Out1/1
  [hmc1_1_data_valid] -> Out2/1

== system s_b4a4x4kf/sys3/vacc/hmc_vacc/hmc_rd_cnt ==
  out_reg : Inport
  assert_reg : xbsIndex_r4/Assert  assert_type=on  type_source=Explicitly  gui_display_data_type=Fixed-point  arith_type=Unsigned  n_bits=32  bin_pt=0  preci_type=Single  exp_width=8  frac_width=24  assert_rate=off  rate_source=Explicitly  period=1  output_port=on  block_type=assert
  cast_gw : xbsIndex_r4/Convert  gui_display_data_type=Fixed-point  arith_type=Unsigned  n_bits=32  bin_pt=0  float_type=Single  exp_bits=8  fraction_bits=24  quantization=Truncate  overflow=Wrap  en=off  latency=1  pipeline=off  dbl_ovrd=off  block_type=convert
  io_delay : xbsIndex_r4/Delay  rst=off  infoeditControl=Selection of Reset will increase slice count due to use of real FFs and instead of SRLs  en=off  latency=0  reg_retiming=on  dbl_ovrd=off  block_type=delay
  reint1 : xbsIndex_r4/Reinterpret  force_arith_type=on  arith_type=Unsigned  force_bin_pt=on  bin_pt=0  block_type=reinterpret
  s_b4a4x4kf_sys3_vacc_hmc_vacc_hmc_rd_cnt_user_data_in : xbsIndex_r4/Gateway Out  inherit_from_input=off  hdl_port=on  rows=1  columns=1  UseAsDAC=off  DACChannel='1'  interface=None  automatic_assignment=on  address_offset=hex2dec('00')  intf_name=''  intf_description=''  timing_constraint=None  locs_specified=off  LOCs={}  io_standard={}  block_type=gatewayout
  sim_out : Terminator
  wires:
  io_delay/1 -> cast_gw/1
  cast_gw/1 -> s_b4a4x4kf_sys3_vacc_hmc_vacc_hmc_rd_cnt_user_data_in/1
  s_b4a4x4kf_sys3_vacc_hmc_vacc_hmc_rd_cnt_user_data_in/1 -> sim_out/1
  out_reg/1 -> assert_reg/1
  assert_reg/1 -> reint1/1
  reint1/1 -> io_delay/1

== system s_b4a4x4kf/sys3/vacc/hmc_vacc/hmc_reord ==
  note: delay rst a bit longer than needed,
      | just in case.
      | HMC won't output valid data for a
      | while after the VACC comes out of reset
  note: clear the valid
      | entries on reset
  rst : Inport
  data_in : Inport  Port=2
  valid_in : Inport  Port=3
  tag_in : Inport  Port=4
  Concat : xbsIndex_r4/Concat  num_inputs=3  dbl_ovrd=off  block_type=concat
  Constant2 : xbsIndex_r4/Constant  const=0  gui_display_data_type=Fixed-point  arith_type=Unsigned  n_bits=266  bin_pt=0  preci_type=Single  exp_width=8  frac_width=24  explicit_period=on  period=1  equ=P=C  opselect=C  inp2=PCIN>>17  opr=+  inp1=P  carry=CIN  dbl_ovrd=off  block_type=constant
  Constant3 : xbsIndex_r4/Constant  const=1  gui_display_data_type=Fixed-point  arith_type=Unsigned  n_bits=1  bin_pt=0  preci_type=Single  exp_width=8  frac_width=24  explicit_period=on  period=1  equ=P=C  opselect=C  inp2=PCIN>>17  opr=+  inp1=P  carry=CIN  dbl_ovrd=off  block_type=constant
  Convert : xbsIndex_r4/Convert  gui_display_data_type=Boolean  arith_type=Boolean  n_bits=1  bin_pt=0  float_type=Single  exp_bits=8  fraction_bits=24  quantization=Truncate  overflow=Wrap  en=off  latency=0  pipeline=off  dbl_ovrd=off  block_type=convert
  Delay1 : xbsIndex_r4/Delay  rst=off  infoeditControl=Selection of Reset will increase slice count due to use of real FFs and instead of SRLs  en=off  latency=2  reg_retiming=off  dbl_ovrd=off  block_type=delay
      settings: infoedit=Hardware notes: A delay line is a chain, each link of which is an SRL16 or SRL32 followed by a flip-flop.
  Delay6 : xbsIndex_r4/Delay  rst=off  infoeditControl=Selection of Reset will increase slice count due to use of real FFs and instead of SRLs  en=off  latency=1  reg_retiming=off  dbl_ovrd=off  block_type=delay
      settings: infoedit=Hardware notes: A delay line is a chain, each link of which is an SRL16 or SRL32 followed by a flip-flop.
  Delay7 : xbsIndex_r4/Delay  rst=off  infoeditControl=Selection of Reset will increase slice count due to use of real FFs and instead of SRLs  en=off  latency=1  reg_retiming=off  dbl_ovrd=off  block_type=delay
      settings: infoedit=Hardware notes: A delay line is a chain, each link of which is an SRL16 or SRL32 followed by a flip-flop.
  Delay8 : xbsIndex_r4/Delay  rst=off  infoeditControl=Selection of Reset will increase slice count due to use of real FFs and instead of SRLs  en=off  latency=1  reg_retiming=off  dbl_ovrd=off  block_type=delay
      settings: infoedit=Hardware notes: A delay line is a chain, each link of which is an SRL16 or SRL32 followed by a flip-flop.
  Delay9 : xbsIndex_r4/Delay  rst=off  infoeditControl=Selection of Reset will increase slice count due to use of real FFs and instead of SRLs  en=off  latency=2  reg_retiming=off  dbl_ovrd=off  block_type=delay
      settings: infoedit=Hardware notes: A delay line is a chain, each link of which is an SRL16 or SRL32 followed by a flip-flop.
  Inverter : xbsIndex_r4/Inverter  en=off  latency=0  dbl_ovrd=off  block_type=inv
  Inverter1 : xbsIndex_r4/Inverter  en=off  latency=0  dbl_ovrd=off  block_type=inv
  Logical : xbsIndex_r4/Logical  logical_function=AND  inputs=2  en=off  latency=0  precision=Full  arith_type=Unsigned  n_bits=16  bin_pt=0  align_bp=on  dbl_ovrd=off  block_type=logical
  Logical1 : xbsIndex_r4/Logical  logical_function=OR  inputs=2  en=off  latency=0  precision=Full  arith_type=Unsigned  n_bits=16  bin_pt=0  align_bp=on  dbl_ovrd=off  block_type=logical
  Logical2 : xbsIndex_r4/Logical  logical_function=OR  inputs=2  en=off  latency=0  precision=Full  arith_type=Unsigned  n_bits=16  bin_pt=0  align_bp=on  dbl_ovrd=off  block_type=logical
  Logical3 : xbsIndex_r4/Logical  logical_function=AND  inputs=2  en=off  latency=0  precision=Full  arith_type=Unsigned  n_bits=16  bin_pt=0  align_bp=on  dbl_ovrd=off  block_type=logical
  Slice1 : xbsIndex_r4/Slice  nbits=256  boolean_output=off  mode=Lower Bit Location + Width  bit1=0  base1=MSB of Input  bit0=9  base0=LSB of Input  dbl_ovrd=off  block_type=slice
      settings: block_version=9.2.01
  Slice11 : xbsIndex_r4/Slice  nbits=9  boolean_output=off  mode=Lower Bit Location + Width  bit1=-1  base1=MSB of Input  bit0=0  base0=LSB of Input  dbl_ovrd=off  block_type=slice
      settings: block_version=9.2.01
  Slice2 : xbsIndex_r4/Slice  nbits=1  boolean_output=off  mode=Upper Bit Location + Width  bit1=0  base1=MSB of Input  bit0=0  base0=LSB of Input  dbl_ovrd=off  block_type=slice
      settings: block_version=9.2.01
  Slice3 : xbsIndex_r4/Slice  nbits=9  boolean_output=off  mode=Lower Bit Location + Width  bit1=-1  base1=MSB of Input  bit0=0  base0=LSB of Input  dbl_ovrd=off  block_type=slice
      settings: block_version=9.2.01
  Slice4 : xbsIndex_r4/Slice  nbits=9  boolean_output=off  mode=Lower Bit Location + Width  bit1=-1  base1=MSB of Input  bit0=0  base0=LSB of Input  dbl_ovrd=off  block_type=slice
      settings: block_version=9.2.01
  Slice5 : xbsIndex_r4/Slice  nbits=256  boolean_output=off  mode=Lower Bit Location + Width  bit1=-1  base1=MSB of Input  bit0=0  base0=LSB of Input  dbl_ovrd=off  block_type=slice
      settings: block_version=9.2.01
  dpr : xbsIndex_r4/Dual Port RAM  depth=512  initVector=0  distributed_mem=Block RAM  init_a=0  init_b=0  rst_a=off  rst_b=off  en_a=off  en_b=off  latency=2  write_mode_A=Read Before Write  write_mode_B=Read Before Write  optimize=Area  dbl_ovrd=off  block_type=dpram
  edge_detect2 : Subsystem  mask(edge_detect){edge=Falling, polarity=Active High, x_in=[0 0.08 0.08 0.16 0.16 0.24 0.24 0.32 0.32 0.4], y_in=[-1 -1  1  1  1  1  1  1  1  1], x_out=[0.6 0.68 0.68 0.76 0.76 0.84 0.84 0.92 0.92 1], y_out=[-1 -1  1  1 -1 -1 -1 -1 -1 -1]}
      mask prompts: edge "Edge Type"; polarity "Output Polarity"; x_in "Input X Positions"; y_in "Input Y Positions"; x_out "Output X Positions"; y_out "Output Y Positions"
      mask help: Output is active for one-cycle after each edge of the specified type (i.e. rising, falling or both).
      mask init: same as s_b4a4x4kf/edge_detect
      settings: AttributesFormatString=|
      | falling edges
      | active high
      mask Help: Output is active for one-cycle after each edge of the specified type (i.e. rising, falling, or both).  Latency is zero.
      mask TypeOptions edge: Rising | Falling | Both
      mask TypeOptions polarity: Active High | Active Low
      mask Display:
      | plot(x_in_num,0.5+y_in_num*0.2);
      | plot(x_out_num,0.5+y_out_num*0.2);
  max_hold : Subsystem
  rd_index : xbsIndex_r4/Counter  cnt_type=Free Running  cnt_to=1  operation=Up  start_count=0  cnt_by_val=1  arith_type=Unsigned  n_bits=9  bin_pt=0  load_pin=off  rst=on  en=on  explicit_period=on  period=1  use_behavioral_HDL=off  implementation=Fabric  use_rpm=off  dbl_ovrd=off  block_type=counter
  run_like_the_wind : Subsystem  mask{window_size=250}
      mask prompts: window_size "randomness gap (words)"
  stutter : Subsystem  mask{latency=2}
      mask prompts: latency "BRAM latency"
  data_out : Outport
  valid_out : Outport  Port=2
  tag_out : Outport  Port=3
  err : Outport  Port=4
  wires:
  valid_in/1 -> [valid_in]
  tag_in/1 -> [tag_in], Slice3/1, Slice11/1
  Slice5/1 -> Concat/2
  data_in/1 -> Slice5/1
  Constant2/1 -> dpr/5
  dpr/2 -> Slice4/1, Slice2/1, Slice1/1
  rd_index/1 -> [rd_idx]
  Slice1/1 -> data_out/1
  Constant3/1 -> Concat/1
  Concat/1 -> dpr/2
  Slice2/1 -> Convert/1
  run_like_the_wind/1(rd_en) -> [run]
  Slice11/1 -> dpr/1, Delay6/1
  Convert/1 -> [mem_valid]
  Delay1/1 -> [valid_out], valid_out/1
  Logical2/1 -> Logical3/1, Logical1/1
  stutter/1(rd) -> [stutter]
  Slice3/1 -> Concat/3
  Slice4/1 -> tag_out/1
  max_hold/1(max) -> [max]
  rst/1 -> Delay7/1
  [rst] -> max_hold/3(rst)
  Delay7/1 -> [rst]
  Delay6/1 -> max_hold/1(value)
  Delay8/1 -> max_hold/2(valid)
  [valid_in] -> Delay8/1
  [valid_in] -> dpr/3
  [max] -> run_like_the_wind/1(max)
  [rd_idx] -> dpr/4
  [rd_idx] -> run_like_the_wind/2(rd_idx)
  [run] -> Logical2/1
  [stutter] -> Logical2/2
  [mem_valid] -> stutter/1(valid_mem)
  Logical/1 -> err/1
  [mem_valid] -> Inverter/1
  [valid_out] -> Logical/1
  Inverter/1 -> Logical/2
  [rst] -> edge_detect2/1(in)
  edge_detect2/1(out) -> rd_index/1
  Logical1/1 -> stutter/2(read_en), dpr/6, rd_index/2
  [rst] -> Logical1/2
  Inverter1/1 -> Logical3/2
  Logical3/1 -> Delay1/1
  [rst] -> Delay9/1
  Delay9/1 -> Inverter1/1
